simulink model "nms_sim_2D_cost"  (R2024b)
settings: Solver=ode15s  StartTime=0.0  StopTime=t_sim  MaxStep=dt_max  EnableMultiTasking=on
values from neighbouring files (symbols this model uses):
  a_BFSH = param_ctrl(35)*1    [setCtrlPar_optim_CPGreflex2001_2D.m]
  a_GAS = param_ctrl(37)*1    [setCtrlPar_optim_CPGreflex2001_2D.m]
  a_GLU = param_ctrl(31)*1    [setCtrlPar_optim_CPGreflex2001_2D.m]
  a_HAM = param_ctrl(33)*1    [setCtrlPar_optim_CPGreflex2001_2D.m]
  a_HFL = param_ctrl(32)*1    [setCtrlPar_optim_CPGreflex2001_2D.m]
  a_RF = param_ctrl(34)*1    [setCtrlPar_optim_CPGreflex2001_2D.m]
  a_SOL = param_ctrl(38)*1    [setCtrlPar_optim_CPGreflex2001_2D.m]
  a_TA = param_ctrl(39)*1    [setCtrlPar_optim_CPGreflex2001_2D.m]
  a_VAS = param_ctrl(36)*1    [setCtrlPar_optim_CPGreflex2001_2D.m]
  ai = param_ctrl(96)*2.0    [setCtrlPar_optim_CPGreflex2001_2D.m]
  b_BFSH = param_ctrl(52)*.51    [setCtrlPar_optim_CPGreflex2001_2D.m]
  b_BFSHGAS = param_ctrl(55)*.51    [setCtrlPar_optim_CPGreflex2001_2D.m]
  b_BFSHHAM = param_ctrl(54)*.51    [setCtrlPar_optim_CPGreflex2001_2D.m]
  b_BFSHVAS = param_ctrl(53)*.51    [setCtrlPar_optim_CPGreflex2001_2D.m]
  b_GAS = param_ctrl(59)*.51    [setCtrlPar_optim_CPGreflex2001_2D.m]
  b_GASBFSH = param_ctrl(60)*.51    [setCtrlPar_optim_CPGreflex2001_2D.m]
  b_GASSOL = param_ctrl(61)*.51    [setCtrlPar_optim_CPGreflex2001_2D.m]
  b_GLU = param_ctrl(40)*.51    [setCtrlPar_optim_CPGreflex2001_2D.m]
  b_GLUHAM = param_ctrl(42)*.51    [setCtrlPar_optim_CPGreflex2001_2D.m]
  b_GLUHFL = param_ctrl(41)*.51    [setCtrlPar_optim_CPGreflex2001_2D.m]
  b_HAM = param_ctrl(46)*.51    [setCtrlPar_optim_CPGreflex2001_2D.m]
  b_HAMBFSH = param_ctrl(48)*.51    [setCtrlPar_optim_CPGreflex2001_2D.m]
  b_HAMGLU = param_ctrl(47)*.51    [setCtrlPar_optim_CPGreflex2001_2D.m]
  b_HFL = param_ctrl(43)*.51    [setCtrlPar_optim_CPGreflex2001_2D.m]
  b_HFLGLU = param_ctrl(44)*.51    [setCtrlPar_optim_CPGreflex2001_2D.m]
  b_HFLRF = param_ctrl(45)*.51    [setCtrlPar_optim_CPGreflex2001_2D.m]
  b_RF = param_ctrl(49)*.51    [setCtrlPar_optim_CPGreflex2001_2D.m]
  b_RFHFL = param_ctrl(50)*.51    [setCtrlPar_optim_CPGreflex2001_2D.m]
  b_RFVAS = param_ctrl(51)*.51    [setCtrlPar_optim_CPGreflex2001_2D.m]
  b_SOL = param_ctrl(62)*.51    [setCtrlPar_optim_CPGreflex2001_2D.m]
  b_SOLGAS = param_ctrl(64)*.51    [setCtrlPar_optim_CPGreflex2001_2D.m]
  b_SOLTA = param_ctrl(63)*.51    [setCtrlPar_optim_CPGreflex2001_2D.m]
  b_TA = param_ctrl(65)*.51    [setCtrlPar_optim_CPGreflex2001_2D.m]
  b_TASOL = param_ctrl(66)*.51    [setCtrlPar_optim_CPGreflex2001_2D.m]
  b_VAS = param_ctrl(56)*.51    [setCtrlPar_optim_CPGreflex2001_2D.m]
  b_VASBFSH = param_ctrl(57)*.51    [setCtrlPar_optim_CPGreflex2001_2D.m]
  b_VASRF = param_ctrl(58)*.51    [setCtrlPar_optim_CPGreflex2001_2D.m]
  bias = param_ctrl(97)*2.5    [setCtrlPar_optim_CPGreflex2001_2D.m]
  c = 0.05    [nms_MS_2D_scaled.m]
  c_jointstop = 0.3 / (pi/180)    (= 17.1887338539)    [nms_MS_2D_scaled.m]
  D12_F = 0.16    *scaleL_JPhys    [nms_MechInit_2D_scaleSkel.m]
  D12_S = 0.2460	*sub_height    [nms_MechInit_2D_scaleSkel.m]
  D12_T = 0.2450  *sub_height    [nms_MechInit_2D_scaleSkel.m]
  D12y_F = 0.039  *sub_height    [nms_MechInit_2D_scaleSkel.m]
  D12z_HAT = 0.1    [nms_MS_2D_scaled.m]
  D13_F = 0.20    *scaleL_JPhys    [nms_MechInit_2D_scaleSkel.m]
  D1G_F = 0.14    *scaleL_JPhys    [nms_MechInit_2D_scaleSkel.m]
  D1G_HAT = 0.35  *scaleL_JPhys    [nms_MechInit_2D_scaleSkel.m]
  D1G_S = (0.3 - D12y_F/4)	*scaleL_JPhys    [nms_MechInit_2D_scaleSkel.m]
  D1G_T = (0.3 - D12y_F/4)	*scaleL_JPhys    [nms_MechInit_2D_scaleSkel.m]
  D1Gy_F = D12y_F*D1G_F/D12_F    (= 0.07)    [nms_MechInit_2D_scaleSkel.m]
  d_BFSH = param_ctrl(26)*1    [setCtrlPar_optim_CPGreflex2001_2D.m]
  d_GAS = param_ctrl(28)*1    [setCtrlPar_optim_CPGreflex2001_2D.m]
  d_GLU = param_ctrl(22)*1    [setCtrlPar_optim_CPGreflex2001_2D.m]
  d_HAM = param_ctrl(24)*1    [setCtrlPar_optim_CPGreflex2001_2D.m]
  d_HFL = param_ctrl(23)*1    [setCtrlPar_optim_CPGreflex2001_2D.m]
  d_RF = param_ctrl(25)*1    [setCtrlPar_optim_CPGreflex2001_2D.m]
  d_SOL = param_ctrl(29)*1    [setCtrlPar_optim_CPGreflex2001_2D.m]
  d_TA = param_ctrl(30)*1    [setCtrlPar_optim_CPGreflex2001_2D.m]
  d_VAS = param_ctrl(27)*1    [setCtrlPar_optim_CPGreflex2001_2D.m]
  DeltaThRef = 5e-3    (= 0.005)    [nms_MS_2D_scaled.m]
  dloptBFSH = 3.0    (= 3)    [setCtrlPar_optim_CPGreflex2001_2D.m]
  dloptGAS = 3.0    (= 3)    [setCtrlPar_optim_CPGreflex2001_2D.m]
  dloptGLU = 3.0    (= 3)    [setCtrlPar_optim_CPGreflex2001_2D.m]
  dloptHAM = 3.0    (= 3)    [setCtrlPar_optim_CPGreflex2001_2D.m]
  dloptHFL = 3.0    (= 3)    [setCtrlPar_optim_CPGreflex2001_2D.m]
  dloptRF = 3.0    (= 3)    [setCtrlPar_optim_CPGreflex2001_2D.m]
  dloptSOL = 3.0    (= 3)    [setCtrlPar_optim_CPGreflex2001_2D.m]
  dloptTA = 3.0    (= 3)    [setCtrlPar_optim_CPGreflex2001_2D.m]
  dloptVAS = 3.0    (= 3)    [setCtrlPar_optim_CPGreflex2001_2D.m]
  ec_BFSH = param_ctrl(80)*0.15    [setCtrlPar_optim_CPGreflex2001_2D.m]
  ec_GAS = param_ctrl(82)*0.15    [setCtrlPar_optim_CPGreflex2001_2D.m]
  ec_GLU = param_ctrl(76)*0.15    [setCtrlPar_optim_CPGreflex2001_2D.m]
  ec_HAM = param_ctrl(78)*0.15    [setCtrlPar_optim_CPGreflex2001_2D.m]
  ec_HFL = param_ctrl(77)*0.15    [setCtrlPar_optim_CPGreflex2001_2D.m]
  ec_RF = param_ctrl(79)*0.15    [setCtrlPar_optim_CPGreflex2001_2D.m]
  ec_TA = param_ctrl(84)*0.15    [setCtrlPar_optim_CPGreflex2001_2D.m]
  ec_VAS = param_ctrl(81)*0.15    [setCtrlPar_optim_CPGreflex2001_2D.m]
  eref = 0.04    [nms_MS_2D_scaled.m]
  eref_GAS = 0.1    [nms_MS_2D_scaled.m]
  eref_SOL = 0.1    [nms_MS_2D_scaled.m]
  es_BFSH = param_ctrl(89)*0.15    [setCtrlPar_optim_CPGreflex2001_2D.m]
  es_GAS = param_ctrl(91)*0.15    [setCtrlPar_optim_CPGreflex2001_2D.m]
  es_GLU = param_ctrl(85)*0.15    [setCtrlPar_optim_CPGreflex2001_2D.m]
  es_HAM = param_ctrl(87)*0.15    [setCtrlPar_optim_CPGreflex2001_2D.m]
  es_HFL = param_ctrl(86)*0.15    [setCtrlPar_optim_CPGreflex2001_2D.m]
  es_RF = param_ctrl(88)*0.15    [setCtrlPar_optim_CPGreflex2001_2D.m]
  es_TA = param_ctrl(93)*0.15    [setCtrlPar_optim_CPGreflex2001_2D.m]
  es_VAS = param_ctrl(90)*0.15    [setCtrlPar_optim_CPGreflex2001_2D.m]
  FmaxBFSH = 350    [nms_MS_2D_scaled.m]
  FmaxGAS = 2000    [nms_MS_2D_scaled.m]
  FmaxGLU = 4000    [nms_MS_2D_scaled.m]
  FmaxHAM = 2000    [nms_MS_2D_scaled.m]
  FmaxHFL = 2000    [nms_MS_2D_scaled.m]
  FmaxRF = 850    [nms_MS_2D_scaled.m]
  FmaxSOL = 4000    [nms_MS_2D_scaled.m]
  FmaxTA = 800    [nms_MS_2D_scaled.m]
  FmaxVAS = 5000    [nms_MS_2D_scaled.m]
  g = 9.81    [nms_MS_2D_scaled.m]
  gamma_4 = param_ctrl(11) * 1.7    [setCtrlPar_optim_CPGreflexsynergy2023_2D.m]
  h_BFSH = param_ctrl(71)*.1    [setCtrlPar_optim_CPGreflex2001_2D.m]
  h_GAS = param_ctrl(73)*.1    [setCtrlPar_optim_CPGreflex2001_2D.m]
  h_GLU = param_ctrl(67)*.1    [setCtrlPar_optim_CPGreflex2001_2D.m]
  h_HAM = param_ctrl(69)*.1    [setCtrlPar_optim_CPGreflex2001_2D.m]
  h_HFL = param_ctrl(68)*.1    [setCtrlPar_optim_CPGreflex2001_2D.m]
  h_RF = param_ctrl(70)*.1    [setCtrlPar_optim_CPGreflex2001_2D.m]
  h_SOL = param_ctrl(74)*.1    [setCtrlPar_optim_CPGreflex2001_2D.m]
  h_TA = param_ctrl(75)*.1    [setCtrlPar_optim_CPGreflex2001_2D.m]
  h_VAS = param_ctrl(72)*.1    [setCtrlPar_optim_CPGreflex2001_2D.m]
  HLCtrlPar = [theta_tgt l_clr alpha_tgt alpha_cd alpha_cv]    [setCtrlPar_optim_reflex2015_2D.m]
  In_F = 0.005    *scaleM*scaleL_JPhys^2    [nms_MechInit_2D_scaleSkel.m]
  In_HAT = 2.5    *scaleM*scaleL_JPhys^2    [nms_MechInit_2D_scaleSkel.m]
  In_S = 0.05     *scaleM*scaleL_JPhys^2    [nms_MechInit_2D_scaleSkel.m]
  In_T = 0.15     *scaleM*scaleL_JPhys^2    [nms_MechInit_2D_scaleSkel.m]
  init_exc = 0.01    [setInitPar_optim_2D.m]
  init_fm = 0.01    [setInitPar_optim_2D.m]
  init_lce = 1    [setInitPar_optim_2D.m]
  init_LCPG = param_ctrl(12) * 0.01    [setCtrlPar_optim_CPGreflexsynergy2023_2D.m]
  init_LStance = 1    [setInitPar_optim_2D.m]
  init_N1 = osc_signal1(phi_off_osc_ind)    [setCtrlPar_optim_CPGreflex2001_2D.m]
  ... (+441 more)
undefined symbols (not defined in the file or in its folder): cost_act_exponent, cost_v_tgt, flag_controller, Newton, nStep_obj, nStep_startKin, Raphson, sgn, SSW_kin, terrain_slope_angle, v_plateS1, X, Y, Z
libraries: nesl_utility x94, sm_lib x90, simulink x28, simulink_extras x12
(part 10 of 20)

== system nms_sim_2D_cost/Cost/joint overextension ==
  L ankle pain lower : Fcn  Expr=u(2) * (u(1)<0)
  L ankle pain upper : Fcn  Expr=u(2) * (u(1)>0)
  L hip pain lower : Fcn  Expr=u(2) * (u(1)<0)
  L hip pain upper : Fcn  Expr=u(2) * (u(1)>0)
  L knee pain lower : Fcn  Expr=u(2) * (u(1)<0)
  L knee pain upper : Fcn  Expr=u(2) * (u(1)>0)
  Mux{1,3,5..11,13..14,16} (12 alike) : Mux  Inputs=2
  Mux15 : Mux  Inputs=12
  R ankle pain lower : Fcn  Expr=u(2) * (u(1)<0)
  R ankle pain upper : Fcn  Expr=u(2) * (u(1)>0)
  R hip Pain Upper : Fcn  Expr=u(2) * (u(1)>0)
  R hip pain lower : Fcn  Expr=u(2) * (u(1)<0)
  R hip pain upper : Fcn  Expr=u(2) * (u(1)>0)
  R knee pain lower : Fcn  Expr=u(2) * (u(1)<0)
  Sum{1,3,5,7..15} (12 alike) : Sum  Inputs=-+|
  knee lim : Constant  Value=P_kneeUpLim
  knee lim10 : Constant  Value=P_hipUpLim
  knee lim11 : Constant  Value=P_ankleUpLim
  knee lim12 : Constant  Value=P_hipLowLim
  knee lim13 : Constant  Value=P_kneeLowLim
  knee lim14 : Constant  Value=P_ankleLowLim
  knee lim2 : Constant  Value=P_hipUpLim
  knee lim4 : Constant  Value=P_ankleUpLim
  knee lim6 : Constant  Value=P_hipLowLim
  knee lim7 : Constant  Value=P_kneeLowLim
  knee lim8 : Constant  Value=P_ankleLowLim
  knee lim9 : Constant  Value=P_kneeUpLim
  pain : Outport
  wires:
  [Rphi23] -> Sum1/2
  knee lim/1 -> Sum1/1
  R hip Pain Upper/1 -> Mux15/3
  Mux10/1 -> R hip Pain Upper/1
  [RHipStop] -> Mux1/2
  Sum1/1 -> Mux10/1
  [RKneeStop] -> Mux10/2
  Mux15/1 -> pain/1
  knee lim2/1 -> Sum3/1
  Mux1/1 -> R hip pain upper/1
  [Rphi34] -> Sum3/2
  Sum3/1 -> Mux1/1
  R hip pain upper/1 -> Mux15/1
  R ankle pain upper/1 -> Mux15/5
  Mux3/1 -> R ankle pain upper/1
  knee lim4/1 -> Sum5/1
  Sum5/1 -> Mux3/1
  [Rphi12] -> Sum5/2
  [RAnkleStop] -> Mux3/2
  R hip pain lower/1 -> Mux15/2
  Sum7/1 -> Mux5/1
  [Rphi34] -> Sum7/2
  Mux5/1 -> R hip pain lower/1
  knee lim6/1 -> Sum7/1
  [RHipStop] -> Mux5/2
  [RKneeStop] -> Mux6/2
  knee lim7/1 -> Sum8/1
  Mux6/1 -> R knee pain lower/1
  [Rphi23] -> Sum8/2
  Sum8/1 -> Mux6/1
  Sum9/1 -> Mux7/1
  [Rphi12] -> Sum9/2
  Mux7/1 -> R ankle pain lower/1
  knee lim8/1 -> Sum9/1
  [RAnkleStop] -> Mux7/2
  R knee pain lower/1 -> Mux15/4
  R ankle pain lower/1 -> Mux15/6
  [LAnkleStop] -> Mux16/2
  knee lim14/1 -> Sum15/1
  Mux16/1 -> L ankle pain lower/1
  [Lphi12] -> Sum15/2
  Sum15/1 -> Mux16/1
  Sum14/1 -> Mux14/1
  [Lphi23] -> Sum14/2
  Mux14/1 -> L knee pain lower/1
  knee lim13/1 -> Sum14/1
  [LKneeStop] -> Mux14/2
  [LHipStop] -> Mux13/2
  knee lim12/1 -> Sum13/1
  Mux13/1 -> L hip pain lower/1
  [Lphi34] -> Sum13/2
  Sum13/1 -> Mux13/1
  [LAnkleStop] -> Mux11/2
  [Lphi12] -> Sum12/2
  Sum12/1 -> Mux11/1
  knee lim11/1 -> Sum12/1
  Mux11/1 -> L ankle pain upper/1
  Sum11/1 -> Mux8/1
  [Lphi34] -> Sum11/2
  Mux8/1 -> L hip pain upper/1
  knee lim10/1 -> Sum11/1
  [LKneeStop] -> Mux9/2
  Sum10/1 -> Mux9/1
  [LHipStop] -> Mux8/2
  Mux9/1 -> L knee pain upper/1
  knee lim9/1 -> Sum10/1
  [Lphi23] -> Sum10/2
  L hip pain upper/1 -> Mux15/7
  L knee pain upper/1 -> Mux15/9
  L knee pain lower/1 -> Mux15/10
  L ankle pain upper/1 -> Mux15/11
  L ankle pain lower/1 -> Mux15/12
  L hip pain lower/1 -> Mux15/8

== system nms_sim_2D_cost/Cost/nStep start ==
  nStep : Inport
  Trigger : TriggerPort  VariantControl=Variant  ZeroCross=off
  nStep_start : Outport  InitialOutput=0
  wires:
  nStep/1 -> nStep_start/1

== system nms_sim_2D_cost/Muscle Actuation/ECC ==
  E : Inport
  Constant : Constant  Value=tau_act
  Constant1 : Constant  Value=tau_deact
  Divide : Product  Inputs=*/
  Integrator : Integrator  InitialCondition=init_exc
  Sum : Sum  Inputs=+-|
  Switch : Switch  Criteria=u2 > Threshold  SaturateOnIntegerOverflow=off  InputSameDT=off
  A : Outport  VectorParamsAs1DForOutWhenUnconnected=off
  wires:
  E/1 -> Sum/1
  Integrator/1 -> A/1, Sum/2  "A"
  Divide/1 -> Integrator/1  "dA"
  Sum/1 -> Divide/1, Switch/2
  Switch/1 -> Divide/2
  Constant/1 -> Switch/1
  Constant1/1 -> Switch/3

== system nms_sim_2D_cost/Muscle Actuation/ECC1 ==
  E : Inport
  Constant : Constant  Value=tau_act
  Constant1 : Constant  Value=tau_deact
  Divide : Product  Inputs=*/
  Integrator : Integrator  InitialCondition=init_exc
  Sum : Sum  Inputs=+-|
  Switch : Switch  Criteria=u2 > Threshold  SaturateOnIntegerOverflow=off  InputSameDT=off
  A : Outport  VectorParamsAs1DForOutWhenUnconnected=off
  wires:
  Constant1/1 -> Switch/3
  Constant/1 -> Switch/1
  Switch/1 -> Divide/2
  Sum/1 -> Switch/2, Divide/1
  Divide/1 -> Integrator/1  "dA"
  Integrator/1 -> Sum/2, A/1  "A"
  E/1 -> Sum/1

== system nms_sim_2D_cost/Muscle Actuation/ECC10 ==
  E : Inport
  Constant : Constant  Value=tau_act
  Constant1 : Constant  Value=tau_deact
  Divide : Product  Inputs=*/
  Integrator : Integrator  InitialCondition=init_exc
  Sum : Sum  Inputs=+-|
  Switch : Switch  Criteria=u2 > Threshold  SaturateOnIntegerOverflow=off  InputSameDT=off
  A : Outport  VectorParamsAs1DForOutWhenUnconnected=off
  wires:
  Constant1/1 -> Switch/3
  Constant/1 -> Switch/1
  Switch/1 -> Divide/2
  Sum/1 -> Switch/2, Divide/1
  Divide/1 -> Integrator/1  "dA"
  Integrator/1 -> Sum/2, A/1  "A"
  E/1 -> Sum/1

== system nms_sim_2D_cost/Muscle Actuation/ECC11 ==
  E : Inport
  Constant : Constant  Value=tau_act
  Constant1 : Constant  Value=tau_deact
  Divide : Product  Inputs=*/
  Integrator : Integrator  InitialCondition=init_exc
  Sum : Sum  Inputs=+-|
  Switch : Switch  Criteria=u2 > Threshold  SaturateOnIntegerOverflow=off  InputSameDT=off
  A : Outport  VectorParamsAs1DForOutWhenUnconnected=off
  wires:
  E/1 -> Sum/1
  Integrator/1 -> A/1, Sum/2  "A"
  Divide/1 -> Integrator/1  "dA"
  Sum/1 -> Divide/1, Switch/2
  Switch/1 -> Divide/2
  Constant/1 -> Switch/1
  Constant1/1 -> Switch/3

== system nms_sim_2D_cost/Muscle Actuation/ECC12 ==
  E : Inport
  Constant : Constant  Value=tau_act
  Constant1 : Constant  Value=tau_deact
  Divide : Product  Inputs=*/
  Integrator : Integrator  InitialCondition=init_exc
  Sum : Sum  Inputs=+-|
  Switch : Switch  Criteria=u2 > Threshold  SaturateOnIntegerOverflow=off  InputSameDT=off
  A : Outport  VectorParamsAs1DForOutWhenUnconnected=off
  wires:
  Constant1/1 -> Switch/3
  Constant/1 -> Switch/1
  Switch/1 -> Divide/2
  Sum/1 -> Switch/2, Divide/1
  Divide/1 -> Integrator/1  "dA"
  Integrator/1 -> Sum/2, A/1  "A"
  E/1 -> Sum/1

== system nms_sim_2D_cost/Muscle Actuation/ECC13 ==
  E : Inport
  Constant : Constant  Value=tau_act
  Constant1 : Constant  Value=tau_deact
  Divide : Product  Inputs=*/
  Integrator : Integrator  InitialCondition=init_exc
  Sum : Sum  Inputs=+-|
  Switch : Switch  Criteria=u2 > Threshold  SaturateOnIntegerOverflow=off  InputSameDT=off
  A : Outport  VectorParamsAs1DForOutWhenUnconnected=off
  wires:
  E/1 -> Sum/1
  Integrator/1 -> A/1, Sum/2  "A"
  Divide/1 -> Integrator/1  "dA"
  Sum/1 -> Divide/1, Switch/2
  Switch/1 -> Divide/2
  Constant/1 -> Switch/1
  Constant1/1 -> Switch/3

== system nms_sim_2D_cost/Muscle Actuation/ECC14 ==
  E : Inport
  Constant : Constant  Value=tau_act
  Constant1 : Constant  Value=tau_deact
  Divide : Product  Inputs=*/
  Integrator : Integrator  InitialCondition=init_exc
  Sum : Sum  Inputs=+-|
  Switch : Switch  Criteria=u2 > Threshold  SaturateOnIntegerOverflow=off  InputSameDT=off
  A : Outport  VectorParamsAs1DForOutWhenUnconnected=off
  wires:
  Constant1/1 -> Switch/3
  Constant/1 -> Switch/1
  Switch/1 -> Divide/2
  Sum/1 -> Switch/2, Divide/1
  Divide/1 -> Integrator/1  "dA"
  Integrator/1 -> Sum/2, A/1  "A"
  E/1 -> Sum/1

== system nms_sim_2D_cost/Muscle Actuation/ECC15 ==
  E : Inport
  Constant : Constant  Value=tau_act
  Constant1 : Constant  Value=tau_deact
  Divide : Product  Inputs=*/
  Integrator : Integrator  InitialCondition=init_exc
  Sum : Sum  Inputs=+-|
  Switch : Switch  Criteria=u2 > Threshold  SaturateOnIntegerOverflow=off  InputSameDT=off
  A : Outport  VectorParamsAs1DForOutWhenUnconnected=off
  wires:
  E/1 -> Sum/1
  Integrator/1 -> A/1, Sum/2  "A"
  Divide/1 -> Integrator/1  "dA"
  Sum/1 -> Divide/1, Switch/2
  Switch/1 -> Divide/2
  Constant/1 -> Switch/1
  Constant1/1 -> Switch/3

== system nms_sim_2D_cost/Muscle Actuation/ECC16 ==
  E : Inport
  Constant : Constant  Value=tau_act
  Constant1 : Constant  Value=tau_deact
  Divide : Product  Inputs=*/
  Integrator : Integrator  InitialCondition=init_exc
  Sum : Sum  Inputs=+-|
  Switch : Switch  Criteria=u2 > Threshold  SaturateOnIntegerOverflow=off  InputSameDT=off
  A : Outport  VectorParamsAs1DForOutWhenUnconnected=off
  wires:
  Constant1/1 -> Switch/3
  Constant/1 -> Switch/1
  Switch/1 -> Divide/2
  Sum/1 -> Switch/2, Divide/1
  Divide/1 -> Integrator/1  "dA"
  Integrator/1 -> Sum/2, A/1  "A"
  E/1 -> Sum/1

== system nms_sim_2D_cost/Muscle Actuation/ECC17 ==
  E : Inport
  Constant : Constant  Value=tau_act
  Constant1 : Constant  Value=tau_deact
  Divide : Product  Inputs=*/
  Integrator : Integrator  InitialCondition=init_exc
  Sum : Sum  Inputs=+-|
  Switch : Switch  Criteria=u2 > Threshold  SaturateOnIntegerOverflow=off  InputSameDT=off
  A : Outport  VectorParamsAs1DForOutWhenUnconnected=off
  wires:
  E/1 -> Sum/1
  Integrator/1 -> A/1, Sum/2  "A"
  Divide/1 -> Integrator/1  "dA"
  Sum/1 -> Divide/1, Switch/2
  Switch/1 -> Divide/2
  Constant/1 -> Switch/1
  Constant1/1 -> Switch/3

== system nms_sim_2D_cost/Muscle Actuation/ECC2 ==
  E : Inport
  Constant : Constant  Value=tau_act
  Constant1 : Constant  Value=tau_deact
  Divide : Product  Inputs=*/
  Integrator : Integrator  InitialCondition=init_exc
  Sum : Sum  Inputs=+-|
  Switch : Switch  Criteria=u2 > Threshold  SaturateOnIntegerOverflow=off  InputSameDT=off
  A : Outport  VectorParamsAs1DForOutWhenUnconnected=off
  wires:
  E/1 -> Sum/1
  Integrator/1 -> A/1, Sum/2  "A"
  Divide/1 -> Integrator/1  "dA"
  Sum/1 -> Divide/1, Switch/2
  Switch/1 -> Divide/2
  Constant/1 -> Switch/1
  Constant1/1 -> Switch/3

== system nms_sim_2D_cost/Muscle Actuation/ECC3 ==
  E : Inport
  Constant : Constant  Value=tau_act
  Constant1 : Constant  Value=tau_deact
  Divide : Product  Inputs=*/
  Integrator : Integrator  InitialCondition=init_exc
  Sum : Sum  Inputs=+-|
  Switch : Switch  Criteria=u2 > Threshold  SaturateOnIntegerOverflow=off  InputSameDT=off
  A : Outport  VectorParamsAs1DForOutWhenUnconnected=off
  wires:
  Constant1/1 -> Switch/3
  Constant/1 -> Switch/1
  Switch/1 -> Divide/2
  Sum/1 -> Switch/2, Divide/1
  Divide/1 -> Integrator/1  "dA"
  Integrator/1 -> Sum/2, A/1  "A"
  E/1 -> Sum/1

== system nms_sim_2D_cost/Muscle Actuation/ECC4 ==
  E : Inport
  Constant : Constant  Value=tau_act
  Constant1 : Constant  Value=tau_deact
  Divide : Product  Inputs=*/
  Integrator : Integrator  InitialCondition=init_exc
  Sum : Sum  Inputs=+-|
  Switch : Switch  Criteria=u2 > Threshold  SaturateOnIntegerOverflow=off  InputSameDT=off
  A : Outport  VectorParamsAs1DForOutWhenUnconnected=off
  wires:
  E/1 -> Sum/1
  Integrator/1 -> A/1, Sum/2  "A"
  Divide/1 -> Integrator/1  "dA"
  Sum/1 -> Divide/1, Switch/2
  Switch/1 -> Divide/2
  Constant/1 -> Switch/1
  Constant1/1 -> Switch/3

== system nms_sim_2D_cost/Muscle Actuation/ECC5 ==
  E : Inport
  Constant : Constant  Value=tau_act
  Constant1 : Constant  Value=tau_deact
  Divide : Product  Inputs=*/
  Integrator : Integrator  InitialCondition=init_exc
  Sum : Sum  Inputs=+-|
  Switch : Switch  Criteria=u2 > Threshold  SaturateOnIntegerOverflow=off  InputSameDT=off
  A : Outport  VectorParamsAs1DForOutWhenUnconnected=off
  wires:
  Constant1/1 -> Switch/3
  Constant/1 -> Switch/1
  Switch/1 -> Divide/2
  Sum/1 -> Switch/2, Divide/1
  Divide/1 -> Integrator/1  "dA"
  Integrator/1 -> Sum/2, A/1  "A"
  E/1 -> Sum/1

== system nms_sim_2D_cost/Muscle Actuation/ECC6 ==
  E : Inport
  Constant : Constant  Value=tau_act
  Constant1 : Constant  Value=tau_deact
  Divide : Product  Inputs=*/
  Integrator : Integrator  InitialCondition=init_exc
  Sum : Sum  Inputs=+-|
  Switch : Switch  Criteria=u2 > Threshold  SaturateOnIntegerOverflow=off  InputSameDT=off
  A : Outport  VectorParamsAs1DForOutWhenUnconnected=off
  wires:
  E/1 -> Sum/1
  Integrator/1 -> A/1, Sum/2  "A"
  Divide/1 -> Integrator/1  "dA"
  Sum/1 -> Divide/1, Switch/2
  Switch/1 -> Divide/2
  Constant/1 -> Switch/1
  Constant1/1 -> Switch/3

== system nms_sim_2D_cost/Muscle Actuation/ECC7 ==
  E : Inport
  Constant : Constant  Value=tau_act
  Constant1 : Constant  Value=tau_deact
  Divide : Product  Inputs=*/
  Integrator : Integrator  InitialCondition=init_exc
  Sum : Sum  Inputs=+-|
  Switch : Switch  Criteria=u2 > Threshold  SaturateOnIntegerOverflow=off  InputSameDT=off
  A : Outport  VectorParamsAs1DForOutWhenUnconnected=off
  wires:
  Constant1/1 -> Switch/3
  Constant/1 -> Switch/1
  Switch/1 -> Divide/2
  Sum/1 -> Switch/2, Divide/1
  Divide/1 -> Integrator/1  "dA"
  Integrator/1 -> Sum/2, A/1  "A"
  E/1 -> Sum/1

== system nms_sim_2D_cost/Muscle Actuation/ECC8 ==
  E : Inport
  Constant : Constant  Value=tau_act
  Constant1 : Constant  Value=tau_deact
  Divide : Product  Inputs=*/
  Integrator : Integrator  InitialCondition=init_exc
  Sum : Sum  Inputs=+-|
  Switch : Switch  Criteria=u2 > Threshold  SaturateOnIntegerOverflow=off  InputSameDT=off
  A : Outport  VectorParamsAs1DForOutWhenUnconnected=off
  wires:
  E/1 -> Sum/1
  Integrator/1 -> A/1, Sum/2  "A"
  Divide/1 -> Integrator/1  "dA"
  Sum/1 -> Divide/1, Switch/2
  Switch/1 -> Divide/2
  Constant/1 -> Switch/1
  Constant1/1 -> Switch/3

== system nms_sim_2D_cost/Muscle Actuation/ECC9 ==
  E : Inport
  Constant : Constant  Value=tau_act
  Constant1 : Constant  Value=tau_deact
  Divide : Product  Inputs=*/
  Integrator : Integrator  InitialCondition=init_exc
  Sum : Sum  Inputs=+-|
  Switch : Switch  Criteria=u2 > Threshold  SaturateOnIntegerOverflow=off  InputSameDT=off
  A : Outport  VectorParamsAs1DForOutWhenUnconnected=off
  wires:
  E/1 -> Sum/1
  Integrator/1 -> A/1, Sum/2  "A"
  Divide/1 -> Integrator/1  "dA"
  Sum/1 -> Divide/1, Switch/2
  Switch/1 -> Divide/2
  Constant/1 -> Switch/1
  Constant1/1 -> Switch/3

== system nms_sim_2D_cost/Muscle Actuation/GLU ==
  note: SOLEUS Muscle-Tendon Dynamics
  note: Excitation Contraction Coupling
  A : Inport
  lmtc [m] : Inport  Port=2
  1 : Product  Inputs=**  InputSameDT=on  SaturateOnIntegerOverflow=on  OutDataTypeStr=Inherit: Same as first input
  1/lslack : Gain  Gain=1/lslackGLU  SaturateOnIntegerOverflow=on  OutDataTypeStr=Inherit: Same as input  ParamDataTypeStr=Inherit: Same as input
  BE force-length relation : Subsystem
  CE force-length relation : Subsystem
  CE inverse force-velocity relation : Subsystem
  Constant : Constant  Value=lslackGLU
  Fmax : Gain  Gain=FmaxGLU  SaturateOnIntegerOverflow=on  OutDataTypeStr=Inherit: Same as input  ParamDataTypeStr=Inherit: Same as input
  Fmax1 : Gain  Gain=FmaxGLU  SaturateOnIntegerOverflow=on  OutDataTypeStr=Inherit: Same as input  ParamDataTypeStr=Inherit: Same as input
  "Fpe = F^*pe * fv " : Product  InputSameDT=on  SaturateOnIntegerOverflow=on  OutDataTypeStr=Inherit: Same as first input
  Fv = Fse / (A*Fce) : Product  Inputs=*/  InputSameDT=on  SaturateOnIntegerOverflow=on  OutDataTypeStr=Inherit: Same as first input
  Integrator : Integrator  InitialConditionSource=external  LowerSaturationLimit=0.05
  PE force-length relation : Subsystem
  SE force-length relation : Subsystem
  Sum : Sum  Inputs=|+-  InputSameDT=on  SaturateOnIntegerOverflow=on  OutDataTypeStr=Inherit: Same as first input
  Sum1 : Sum  Inputs=|+-  InputSameDT=on  SaturateOnIntegerOverflow=on  OutDataTypeStr=Inherit: Same as first input
  Sum2 : Sum  Inputs=|-+  InputSameDT=on  SaturateOnIntegerOverflow=on  OutDataTypeStr=Inherit: Same as first input
  Sum3 : Sum  InputSameDT=on  SaturateOnIntegerOverflow=on  OutDataTypeStr=Inherit: Same as first input
  Sum4 : Sum  InputSameDT=on  SaturateOnIntegerOverflow=on  OutDataTypeStr=Inherit: Same as first input
  lce/lopt : Gain  Gain=1/loptGLU  SaturateOnIntegerOverflow=on  OutDataTypeStr=Inherit: Same as input  ParamDataTypeStr=Inherit: Same as input
  vmax*lopt : Gain  Gain=vmaxGLU*loptGLU  SaturateOnIntegerOverflow=on  OutDataTypeStr=Inherit: Same as input  ParamDataTypeStr=Inherit: Same as input
  Fmtc : Outport  InitialOutput=0  VectorParamsAs1DForOutWhenUnconnected=off
  Lce : Outport  Port=2  InitialOutput=0  VectorParamsAs1DForOutWhenUnconnected=off
  Vce : Outport  Port=3  InitialOutput=0  VectorParamsAs1DForOutWhenUnconnected=off
  Fce : Outport  Port=4  InitialOutput=0  VectorParamsAs1DForOutWhenUnconnected=off
  lse [m] : Outport  Port=5  InitialOutput=0  VectorParamsAs1DForOutWhenUnconnected=off
  wires:
  Integrator/1 -> Sum/2, lce/lopt/1, Lce/1  "lce"
  Sum/1 -> lse [m]/1, 1/lslack/1  "lse"
  lce/lopt/1 -> CE force-length relation/1(lce [lopt]), BE force-length relation/1(lce [lopt]), PE force-length relation/1(lce [lopt])
  Fv = Fse / (A*Fce)/1 -> CE inverse force-velocity relation/1(Fv[Fmax]), "Fpe = F^*pe * fv "/1  "fv"
  vmax*lopt/1 -> Integrator/1, Vce/1  "vce"
  lmtc [m]/1 -> Sum2/2, Sum/1  "lmtc"
  Fmax/1 -> Fmtc/1  "Fmtc"
  1/lslack/1 -> SE force-length relation/1(lse [lslack])
  SE force-length relation/1(fse [Fmax]) -> Fmax/1, Sum4/1
  Sum2/1 -> Integrator/2
  Constant/1 -> Sum2/1
  CE force-length relation/1(fce [Fmax]) -> 1/1
  Sum4/1 -> Fv = Fse / (A*Fce)/1, Sum1/1  "Fse+Fbe"
  PE force-length relation/1(fpe [Fmax]) -> Sum3/1, "Fpe = F^*pe * fv "/2
  1/1 -> Sum3/2
  BE force-length relation/1(fbe [Fmax]) -> Sum4/2
  Sum3/1 -> Fv = Fse / (A*Fce)/2
  CE inverse force-velocity relation/1(v[vmax]) -> vmax*lopt/1
  A/1 -> 1/2
  "Fpe = F^*pe * fv "/1 -> Sum1/2
  Sum1/1 -> Fmax1/1  "Fse+Fbe-Fpe"
  Fmax1/1 -> Fce/1

== system nms_sim_2D_cost/Muscle Actuation/GLU Link ==
  note: GLUTEUS Attachment
  phi34 [rad] : Inport
  Constant : Constant  Value=lslackGLU+loptGLU
  Constant1 : Constant  Value=rGLU
  Constant2 : Constant  Value=phirefGLU
  Gain2 : Gain  Gain=rhoGLU
  Product : Product  RndMeth=Zero
  Sum2 : Sum  Inputs=|+-
  Sum5 : Sum  Inputs=|+-
  lmtu [m] : Outport  VectorParamsAs1DForOutWhenUnconnected=off
  lever [m] : Outport  Port=2  VectorParamsAs1DForOutWhenUnconnected=off
  wires:
  Constant/1 -> Sum5/1
  Sum5/1 -> lmtu [m]/1
  Product/1 -> Gain2/1
  phi34 [rad]/1 -> Sum2/1
  Constant2/1 -> Sum2/2
  Sum2/1 -> Product/1
  Constant1/1 -> Product/2, lever [m]/1
  Gain2/1 -> Sum5/2

== system nms_sim_2D_cost/Muscle Actuation/GLU1 ==
  note: SOLEUS Muscle-Tendon Dynamics
  note: Excitation Contraction Coupling
  A : Inport
  lmtc [m] : Inport  Port=2
  1 : Product  Inputs=**  InputSameDT=on  SaturateOnIntegerOverflow=on  OutDataTypeStr=Inherit: Same as first input
  1/lslack : Gain  Gain=1/lslackGLU  SaturateOnIntegerOverflow=on  OutDataTypeStr=Inherit: Same as input  ParamDataTypeStr=Inherit: Same as input
  BE force-length relation : Subsystem
  CE force-length relation : Subsystem
  CE inverse force-velocity relation : Subsystem
  Constant : Constant  Value=lslackGLU
  Fmax : Gain  Gain=FmaxGLU  SaturateOnIntegerOverflow=on  OutDataTypeStr=Inherit: Same as input  ParamDataTypeStr=Inherit: Same as input
  Fmax1 : Gain  Gain=FmaxGLU  SaturateOnIntegerOverflow=on  OutDataTypeStr=Inherit: Same as input  ParamDataTypeStr=Inherit: Same as input
  "Fpe = F^*pe * fv " : Product  InputSameDT=on  SaturateOnIntegerOverflow=on  OutDataTypeStr=Inherit: Same as first input
  Fv = Fse / (A*Fce) : Product  Inputs=*/  InputSameDT=on  SaturateOnIntegerOverflow=on  OutDataTypeStr=Inherit: Same as first input
  Integrator : Integrator  InitialConditionSource=external  LowerSaturationLimit=0.05
  PE force-length relation : Subsystem
  SE force-length relation : Subsystem
  Sum : Sum  Inputs=|+-  InputSameDT=on  SaturateOnIntegerOverflow=on  OutDataTypeStr=Inherit: Same as first input
  Sum1 : Sum  Inputs=|+-  InputSameDT=on  SaturateOnIntegerOverflow=on  OutDataTypeStr=Inherit: Same as first input
  Sum2 : Sum  Inputs=|-+  InputSameDT=on  SaturateOnIntegerOverflow=on  OutDataTypeStr=Inherit: Same as first input
  Sum3 : Sum  InputSameDT=on  SaturateOnIntegerOverflow=on  OutDataTypeStr=Inherit: Same as first input
  Sum4 : Sum  InputSameDT=on  SaturateOnIntegerOverflow=on  OutDataTypeStr=Inherit: Same as first input
  lce/lopt : Gain  Gain=1/loptGLU  SaturateOnIntegerOverflow=on  OutDataTypeStr=Inherit: Same as input  ParamDataTypeStr=Inherit: Same as input
  vmax*lopt : Gain  Gain=vmaxGLU*loptGLU  SaturateOnIntegerOverflow=on  OutDataTypeStr=Inherit: Same as input  ParamDataTypeStr=Inherit: Same as input
  Fmtc : Outport  InitialOutput=0  VectorParamsAs1DForOutWhenUnconnected=off
  Lce : Outport  Port=2  InitialOutput=0  VectorParamsAs1DForOutWhenUnconnected=off
  Vce : Outport  Port=3  InitialOutput=0  VectorParamsAs1DForOutWhenUnconnected=off
  Fce : Outport  Port=4  InitialOutput=0  VectorParamsAs1DForOutWhenUnconnected=off
  lse [m] : Outport  Port=5  InitialOutput=0  VectorParamsAs1DForOutWhenUnconnected=off
  wires:
  Integrator/1 -> Sum/2, lce/lopt/1, Lce/1  "lce"
  lce/lopt/1 -> CE force-length relation/1(lce [lopt]), PE force-length relation/1(lce [lopt]), BE force-length relation/1(lce [lopt])
  Fv = Fse / (A*Fce)/1 -> "Fpe = F^*pe * fv "/1, CE inverse force-velocity relation/1(Fv[Fmax])  "fv"
  vmax*lopt/1 -> Integrator/1, Vce/1  "vce"
  lmtc [m]/1 -> Sum2/2, Sum/1  "lmtc"
  Fmax/1 -> Fmtc/1  "Fmtc"
  1/lslack/1 -> SE force-length relation/1(lse [lslack])
  SE force-length relation/1(fse [Fmax]) -> Fmax/1, Sum4/1
  Sum2/1 -> Integrator/2
  Constant/1 -> Sum2/1
  CE force-length relation/1(fce [Fmax]) -> 1/1
  PE force-length relation/1(fpe [Fmax]) -> "Fpe = F^*pe * fv "/2, Sum3/1
  1/1 -> Sum3/2
  BE force-length relation/1(fbe [Fmax]) -> Sum4/2
  Sum3/1 -> Fv = Fse / (A*Fce)/2
  CE inverse force-velocity relation/1(v[vmax]) -> vmax*lopt/1
  A/1 -> 1/2
  Sum4/1 -> Sum1/1, Fv = Fse / (A*Fce)/1  "Fse+Fbe"
  "Fpe = F^*pe * fv "/1 -> Sum1/2
  Sum1/1 -> Fmax1/1  "Fse+Fbe-Fpe"
  Fmax1/1 -> Fce/1
  Sum/1 -> lse [m]/1, 1/lslack/1  "lse"

== system nms_sim_2D_cost/Muscle Actuation/HAM ==
  note: SOLEUS Muscle-Tendon Dynamics
  note: Excitation Contraction Coupling
  A : Inport
  lmtc [m] : Inport  Port=2
  1 : Product  Inputs=**  InputSameDT=on  SaturateOnIntegerOverflow=on  OutDataTypeStr=Inherit: Same as first input
  1/lslack : Gain  Gain=1/lslackHAM  SaturateOnIntegerOverflow=on  OutDataTypeStr=Inherit: Same as input  ParamDataTypeStr=Inherit: Same as input
  BE force-length relation : Subsystem
  CE force-length relation : Subsystem
  CE inverse force-velocity relation : Subsystem
  Constant : Constant  Value=lslackHAM
  Fmax : Gain  Gain=FmaxHAM  SaturateOnIntegerOverflow=on  OutDataTypeStr=Inherit: Same as input  ParamDataTypeStr=Inherit: Same as input
  Fmax1 : Gain  Gain=FmaxHAM  SaturateOnIntegerOverflow=on  OutDataTypeStr=Inherit: Same as input  ParamDataTypeStr=Inherit: Same as input
  "Fpe = F^*pe * fv " : Product  InputSameDT=on  SaturateOnIntegerOverflow=on  OutDataTypeStr=Inherit: Same as first input
  Fv = Fse / (A*Fce) : Product  Inputs=*/  InputSameDT=on  SaturateOnIntegerOverflow=on  OutDataTypeStr=Inherit: Same as first input
  Integrator : Integrator  InitialConditionSource=external  LowerSaturationLimit=0.05
  PE force-length relation : Subsystem
  SE force-length relation : Subsystem
  Sum : Sum  Inputs=|+-  InputSameDT=on  SaturateOnIntegerOverflow=on  OutDataTypeStr=Inherit: Same as first input
  Sum1 : Sum  Inputs=|+-  InputSameDT=on  SaturateOnIntegerOverflow=on  OutDataTypeStr=Inherit: Same as first input
  Sum2 : Sum  Inputs=|-+  InputSameDT=on  SaturateOnIntegerOverflow=on  OutDataTypeStr=Inherit: Same as first input
  Sum3 : Sum  InputSameDT=on  SaturateOnIntegerOverflow=on  OutDataTypeStr=Inherit: Same as first input
  Sum4 : Sum  InputSameDT=on  SaturateOnIntegerOverflow=on  OutDataTypeStr=Inherit: Same as first input
  lce/lopt : Gain  Gain=1/loptHAM  SaturateOnIntegerOverflow=on  OutDataTypeStr=Inherit: Same as input  ParamDataTypeStr=Inherit: Same as input
  vmax*lopt : Gain  Gain=vmaxHAM*loptHAM  SaturateOnIntegerOverflow=on  OutDataTypeStr=Inherit: Same as input  ParamDataTypeStr=Inherit: Same as input
  Fmtc : Outport  InitialOutput=0  VectorParamsAs1DForOutWhenUnconnected=off
  Lce : Outport  Port=2  InitialOutput=0  VectorParamsAs1DForOutWhenUnconnected=off
  Vce : Outport  Port=3  InitialOutput=0  VectorParamsAs1DForOutWhenUnconnected=off
  Fce : Outport  Port=4  InitialOutput=0  VectorParamsAs1DForOutWhenUnconnected=off
  lse [m] : Outport  Port=5  InitialOutput=0  VectorParamsAs1DForOutWhenUnconnected=off
  wires:
  Integrator/1 -> Sum/2, lce/lopt/1, Lce/1  "lce"
  lce/lopt/1 -> CE force-length relation/1(lce [lopt]), PE force-length relation/1(lce [lopt]), BE force-length relation/1(lce [lopt])
  Fv = Fse / (A*Fce)/1 -> "Fpe = F^*pe * fv "/1, CE inverse force-velocity relation/1(Fv[Fmax])  "fv"
  vmax*lopt/1 -> Integrator/1, Vce/1  "vce"
  lmtc [m]/1 -> Sum2/2, Sum/1  "lmtc"
  Fmax/1 -> Fmtc/1  "Fmtc"
  1/lslack/1 -> SE force-length relation/1(lse [lslack])
  SE force-length relation/1(fse [Fmax]) -> Fmax/1, Sum4/1
  Sum2/1 -> Integrator/2
  Constant/1 -> Sum2/1
  CE force-length relation/1(fce [Fmax]) -> 1/1
  PE force-length relation/1(fpe [Fmax]) -> "Fpe = F^*pe * fv "/2, Sum3/1
  1/1 -> Sum3/2
  BE force-length relation/1(fbe [Fmax]) -> Sum4/2
  Sum3/1 -> Fv = Fse / (A*Fce)/2
  CE inverse force-velocity relation/1(v[vmax]) -> vmax*lopt/1
  A/1 -> 1/2
  Sum4/1 -> Sum1/1, Fv = Fse / (A*Fce)/1  "Fse+Fbe"
  "Fpe = F^*pe * fv "/1 -> Sum1/2
  Sum1/1 -> Fmax1/1  "Fse+Fbe-Fpe"
  Fmax1/1 -> Fce/1
  Sum/1 -> lse [m]/1, 1/lslack/1  "lse"

== system nms_sim_2D_cost/Muscle Actuation/HAM Link ==
  note: HAM Attachment
  phi34 [rad] : Inport
  phi23 [rad] : Inport  Port=2
  Constant1 : Constant  Value=rHAMk
  Constant2 : Constant  Value=phirefHAMk
  Constant3 : Constant  Value=rHAMh
  Constant4 : Constant  Value=lslackHAM+loptHAM
  Constant5 : Constant  Value=phirefHAMh
  Gain2 : Gain  Gain=rhoHAMh
  Gain4 : Gain  Gain=rhoHAMk
  Product : Product  RndMeth=Zero
  Product1 : Product  RndMeth=Zero
  Sum1 : Sum  Inputs=|+-
  Sum4 : Sum  Inputs=|+-
  Sum5 : Sum  Inputs=-++
  lmtu [m] : Outport  VectorParamsAs1DForOutWhenUnconnected=off
  lever34 [m] : Outport  Port=2  VectorParamsAs1DForOutWhenUnconnected=off
  lever23 [m] : Outport  Port=3  VectorParamsAs1DForOutWhenUnconnected=off
  wires:
  Sum5/1 -> lmtu [m]/1
  Constant4/1 -> Sum5/2
  Gain4/1 -> Sum5/3
  Gain2/1 -> Sum5/1
  phi34 [rad]/1 -> Sum4/1
  Constant5/1 -> Sum4/2
  Sum4/1 -> Product/1
  Constant3/1 -> Product/2, lever34 [m]/1
  Product/1 -> Gain2/1
  phi23 [rad]/1 -> Sum1/1
  Constant2/1 -> Sum1/2
  Sum1/1 -> Product1/1
  Constant1/1 -> Product1/2, lever23 [m]/1
  Product1/1 -> Gain4/1

== system nms_sim_2D_cost/Muscle Actuation/HAM1 ==
  note: SOLEUS Muscle-Tendon Dynamics
  note: Excitation Contraction Coupling
  A : Inport
  lmtc [m] : Inport  Port=2
  1 : Product  Inputs=**  InputSameDT=on  SaturateOnIntegerOverflow=on  OutDataTypeStr=Inherit: Same as first input
  1/lslack : Gain  Gain=1/lslackHAM  SaturateOnIntegerOverflow=on  OutDataTypeStr=Inherit: Same as input  ParamDataTypeStr=Inherit: Same as input
  BE force-length relation : Subsystem
  CE force-length relation : Subsystem
  CE inverse force-velocity relation : Subsystem
  Constant : Constant  Value=lslackHAM
  Fmax : Gain  Gain=FmaxHAM  SaturateOnIntegerOverflow=on  OutDataTypeStr=Inherit: Same as input  ParamDataTypeStr=Inherit: Same as input
  Fmax1 : Gain  Gain=FmaxHAM  SaturateOnIntegerOverflow=on  OutDataTypeStr=Inherit: Same as input  ParamDataTypeStr=Inherit: Same as input
  "Fpe = F^*pe * fv " : Product  InputSameDT=on  SaturateOnIntegerOverflow=on  OutDataTypeStr=Inherit: Same as first input
  Fv = Fse / (A*Fce) : Product  Inputs=*/  InputSameDT=on  SaturateOnIntegerOverflow=on  OutDataTypeStr=Inherit: Same as first input
  Integrator : Integrator  InitialConditionSource=external  LowerSaturationLimit=0.05
  PE force-length relation : Subsystem
  SE force-length relation : Subsystem
  Sum : Sum  Inputs=|+-  InputSameDT=on  SaturateOnIntegerOverflow=on  OutDataTypeStr=Inherit: Same as first input
  Sum1 : Sum  Inputs=|+-  InputSameDT=on  SaturateOnIntegerOverflow=on  OutDataTypeStr=Inherit: Same as first input
  Sum2 : Sum  Inputs=|-+  InputSameDT=on  SaturateOnIntegerOverflow=on  OutDataTypeStr=Inherit: Same as first input
  Sum3 : Sum  InputSameDT=on  SaturateOnIntegerOverflow=on  OutDataTypeStr=Inherit: Same as first input
  Sum4 : Sum  InputSameDT=on  SaturateOnIntegerOverflow=on  OutDataTypeStr=Inherit: Same as first input
  lce/lopt : Gain  Gain=1/loptHAM  SaturateOnIntegerOverflow=on  OutDataTypeStr=Inherit: Same as input  ParamDataTypeStr=Inherit: Same as input
  vmax*lopt : Gain  Gain=vmaxHAM*loptHAM  SaturateOnIntegerOverflow=on  OutDataTypeStr=Inherit: Same as input  ParamDataTypeStr=Inherit: Same as input
  Fmtc : Outport  InitialOutput=0  VectorParamsAs1DForOutWhenUnconnected=off
  Lce : Outport  Port=2  InitialOutput=0  VectorParamsAs1DForOutWhenUnconnected=off
  Vce : Outport  Port=3  InitialOutput=0  VectorParamsAs1DForOutWhenUnconnected=off
  Fce : Outport  Port=4  InitialOutput=0  VectorParamsAs1DForOutWhenUnconnected=off
  lse [m] : Outport  Port=5  InitialOutput=0  VectorParamsAs1DForOutWhenUnconnected=off
  wires:
  Integrator/1 -> Sum/2, lce/lopt/1, Lce/1  "lce"
  lce/lopt/1 -> CE force-length relation/1(lce [lopt]), PE force-length relation/1(lce [lopt]), BE force-length relation/1(lce [lopt])
  Fv = Fse / (A*Fce)/1 -> "Fpe = F^*pe * fv "/1, CE inverse force-velocity relation/1(Fv[Fmax])  "fv"
  vmax*lopt/1 -> Integrator/1, Vce/1  "vce"
  lmtc [m]/1 -> Sum2/2, Sum/1  "lmtc"
  Fmax/1 -> Fmtc/1  "Fmtc"
  1/lslack/1 -> SE force-length relation/1(lse [lslack])
  SE force-length relation/1(fse [Fmax]) -> Fmax/1, Sum4/1
  Sum2/1 -> Integrator/2
  Constant/1 -> Sum2/1
  CE force-length relation/1(fce [Fmax]) -> 1/1
  PE force-length relation/1(fpe [Fmax]) -> "Fpe = F^*pe * fv "/2, Sum3/1
  1/1 -> Sum3/2
  BE force-length relation/1(fbe [Fmax]) -> Sum4/2
  Sum3/1 -> Fv = Fse / (A*Fce)/2
  CE inverse force-velocity relation/1(v[vmax]) -> vmax*lopt/1
  A/1 -> 1/2
  Sum4/1 -> Sum1/1, Fv = Fse / (A*Fce)/1  "Fse+Fbe"
  "Fpe = F^*pe * fv "/1 -> Sum1/2
  Sum1/1 -> Fmax1/1  "Fse+Fbe-Fpe"
  Fmax1/1 -> Fce/1
  Sum/1 -> lse [m]/1, 1/lslack/1  "lse"

== system nms_sim_2D_cost/Muscle Actuation/HFL ==
  note: SOLEUS Muscle-Tendon Dynamics
  note: Excitation Contraction Coupling
  A : Inport
  lmtc [m] : Inport  Port=2
  1 : Product  Inputs=**  InputSameDT=on  SaturateOnIntegerOverflow=on  OutDataTypeStr=Inherit: Same as first input
  1/lslack : Gain  Gain=1/lslackHFL  SaturateOnIntegerOverflow=on  OutDataTypeStr=Inherit: Same as input  ParamDataTypeStr=Inherit: Same as input
  BE force-length relation : Subsystem
  CE force-length relation : Subsystem
  CE inverse force-velocity relation : Subsystem
  Constant : Constant  Value=lslackHFL
  Fmax : Gain  Gain=FmaxHFL  SaturateOnIntegerOverflow=on  OutDataTypeStr=Inherit: Same as input  ParamDataTypeStr=Inherit: Same as input
  Fmax1 : Gain  Gain=FmaxHFL  SaturateOnIntegerOverflow=on  OutDataTypeStr=Inherit: Same as input  ParamDataTypeStr=Inherit: Same as input
  "Fpe = F^*pe * fv " : Product  InputSameDT=on  SaturateOnIntegerOverflow=on  OutDataTypeStr=Inherit: Same as first input
  Fv = Fse / (A*Fce) : Product  Inputs=*/  InputSameDT=on  SaturateOnIntegerOverflow=on  OutDataTypeStr=Inherit: Same as first input
  Integrator : Integrator  InitialConditionSource=external  LowerSaturationLimit=0.05
  PE force-length relation : Subsystem
  SE force-length relation : Subsystem
  Sum : Sum  Inputs=|+-  InputSameDT=on  SaturateOnIntegerOverflow=on  OutDataTypeStr=Inherit: Same as first input
  Sum1 : Sum  Inputs=|+-  InputSameDT=on  SaturateOnIntegerOverflow=on  OutDataTypeStr=Inherit: Same as first input
  Sum2 : Sum  Inputs=|-+  InputSameDT=on  SaturateOnIntegerOverflow=on  OutDataTypeStr=Inherit: Same as first input
  Sum3 : Sum  InputSameDT=on  SaturateOnIntegerOverflow=on  OutDataTypeStr=Inherit: Same as first input
  Sum4 : Sum  InputSameDT=on  SaturateOnIntegerOverflow=on  OutDataTypeStr=Inherit: Same as first input
  lce/lopt : Gain  Gain=1/loptHFL  SaturateOnIntegerOverflow=on  OutDataTypeStr=Inherit: Same as input  ParamDataTypeStr=Inherit: Same as input
  vmax*lopt : Gain  Gain=vmaxHFL*loptHFL  SaturateOnIntegerOverflow=on  OutDataTypeStr=Inherit: Same as input  ParamDataTypeStr=Inherit: Same as input
  Fmtc : Outport  InitialOutput=0  VectorParamsAs1DForOutWhenUnconnected=off
  Lce : Outport  Port=2  InitialOutput=0  VectorParamsAs1DForOutWhenUnconnected=off
  Vce : Outport  Port=3  InitialOutput=0  VectorParamsAs1DForOutWhenUnconnected=off
  Fce : Outport  Port=4  InitialOutput=0  VectorParamsAs1DForOutWhenUnconnected=off
  lse [m] : Outport  Port=5  InitialOutput=0  VectorParamsAs1DForOutWhenUnconnected=off
  wires:
  Integrator/1 -> Sum/2, lce/lopt/1, Lce/1  "lce"
  lce/lopt/1 -> CE force-length relation/1(lce [lopt]), PE force-length relation/1(lce [lopt]), BE force-length relation/1(lce [lopt])
  Fv = Fse / (A*Fce)/1 -> "Fpe = F^*pe * fv "/1, CE inverse force-velocity relation/1(Fv[Fmax])  "fv"
  vmax*lopt/1 -> Integrator/1, Vce/1  "vce"
  lmtc [m]/1 -> Sum2/2, Sum/1  "lmtc"
  Fmax/1 -> Fmtc/1  "Fmtc"
  1/lslack/1 -> SE force-length relation/1(lse [lslack])
  SE force-length relation/1(fse [Fmax]) -> Fmax/1, Sum4/1
  Sum2/1 -> Integrator/2
  Constant/1 -> Sum2/1
  CE force-length relation/1(fce [Fmax]) -> 1/1
  PE force-length relation/1(fpe [Fmax]) -> "Fpe = F^*pe * fv "/2, Sum3/1
  1/1 -> Sum3/2
  BE force-length relation/1(fbe [Fmax]) -> Sum4/2
  Sum3/1 -> Fv = Fse / (A*Fce)/2
  CE inverse force-velocity relation/1(v[vmax]) -> vmax*lopt/1
  A/1 -> 1/2
  Sum4/1 -> Sum1/1, Fv = Fse / (A*Fce)/1  "Fse+Fbe"
  "Fpe = F^*pe * fv "/1 -> Sum1/2
  Sum1/1 -> Fmax1/1  "Fse+Fbe-Fpe"
  Fmax1/1 -> Fce/1
  Sum/1 -> lse [m]/1, 1/lslack/1  "lse"

== system nms_sim_2D_cost/Muscle Actuation/HFL Link ==
  note: HFL Attachment
  phi34 [rad] : Inport
  Constant : Constant  Value=lslackHFL+loptHFL
  Constant1 : Constant  Value=rHFL
  Constant2 : Constant  Value=phirefHFL
  Gain2 : Gain  Gain=rhoHFL
  Product : Product  RndMeth=Zero
  Sum2 : Sum  Inputs=|+-
  Sum5 : Sum  Inputs=|++
  lmtu [m] : Outport  VectorParamsAs1DForOutWhenUnconnected=off
  lever [m] : Outport  Port=2  VectorParamsAs1DForOutWhenUnconnected=off
  wires:
  Constant/1 -> Sum5/1
  Sum5/1 -> lmtu [m]/1
  Product/1 -> Gain2/1
  phi34 [rad]/1 -> Sum2/1
  Constant2/1 -> Sum2/2
  Sum2/1 -> Product/1
  Constant1/1 -> Product/2, lever [m]/1
  Gain2/1 -> Sum5/2

== system nms_sim_2D_cost/Muscle Actuation/HFL1 ==
  note: SOLEUS Muscle-Tendon Dynamics
  note: Excitation Contraction Coupling
  A : Inport
  lmtc [m] : Inport  Port=2
  1 : Product  Inputs=**  InputSameDT=on  SaturateOnIntegerOverflow=on  OutDataTypeStr=Inherit: Same as first input
  1/lslack : Gain  Gain=1/lslackHFL  SaturateOnIntegerOverflow=on  OutDataTypeStr=Inherit: Same as input  ParamDataTypeStr=Inherit: Same as input
  BE force-length relation : Subsystem
  CE force-length relation : Subsystem
  CE inverse force-velocity relation : Subsystem
  Constant : Constant  Value=lslackHFL
  Fmax : Gain  Gain=FmaxHFL  SaturateOnIntegerOverflow=on  OutDataTypeStr=Inherit: Same as input  ParamDataTypeStr=Inherit: Same as input
  Fmax1 : Gain  Gain=FmaxHFL  SaturateOnIntegerOverflow=on  OutDataTypeStr=Inherit: Same as input  ParamDataTypeStr=Inherit: Same as input
  "Fpe = F^*pe * fv " : Product  InputSameDT=on  SaturateOnIntegerOverflow=on  OutDataTypeStr=Inherit: Same as first input
  Fv = Fse / (A*Fce) : Product  Inputs=*/  InputSameDT=on  SaturateOnIntegerOverflow=on  OutDataTypeStr=Inherit: Same as first input
  Integrator : Integrator  InitialConditionSource=external  LowerSaturationLimit=0.05
  PE force-length relation : Subsystem
  SE force-length relation : Subsystem
  Sum : Sum  Inputs=|+-  InputSameDT=on  SaturateOnIntegerOverflow=on  OutDataTypeStr=Inherit: Same as first input
  Sum1 : Sum  Inputs=|+-  InputSameDT=on  SaturateOnIntegerOverflow=on  OutDataTypeStr=Inherit: Same as first input
  Sum2 : Sum  Inputs=|-+  InputSameDT=on  SaturateOnIntegerOverflow=on  OutDataTypeStr=Inherit: Same as first input
  Sum3 : Sum  InputSameDT=on  SaturateOnIntegerOverflow=on  OutDataTypeStr=Inherit: Same as first input
  Sum4 : Sum  InputSameDT=on  SaturateOnIntegerOverflow=on  OutDataTypeStr=Inherit: Same as first input
  lce/lopt : Gain  Gain=1/loptHFL  SaturateOnIntegerOverflow=on  OutDataTypeStr=Inherit: Same as input  ParamDataTypeStr=Inherit: Same as input
  vmax*lopt : Gain  Gain=vmaxHFL*loptHFL  SaturateOnIntegerOverflow=on  OutDataTypeStr=Inherit: Same as input  ParamDataTypeStr=Inherit: Same as input
  Fmtc : Outport  InitialOutput=0  VectorParamsAs1DForOutWhenUnconnected=off
  Lce : Outport  Port=2  InitialOutput=0  VectorParamsAs1DForOutWhenUnconnected=off
  Vce : Outport  Port=3  InitialOutput=0  VectorParamsAs1DForOutWhenUnconnected=off
  Fce : Outport  Port=4  InitialOutput=0  VectorParamsAs1DForOutWhenUnconnected=off
  lse [m] : Outport  Port=5  InitialOutput=0  VectorParamsAs1DForOutWhenUnconnected=off
  wires:
  Integrator/1 -> Sum/2, lce/lopt/1, Lce/1  "lce"
  Sum/1 -> lse [m]/1, 1/lslack/1  "lse"
  lce/lopt/1 -> CE force-length relation/1(lce [lopt]), PE force-length relation/1(lce [lopt]), BE force-length relation/1(lce [lopt])
  Fv = Fse / (A*Fce)/1 -> "Fpe = F^*pe * fv "/1, CE inverse force-velocity relation/1(Fv[Fmax])  "fv"
  vmax*lopt/1 -> Integrator/1, Vce/1  "vce"
  lmtc [m]/1 -> Sum2/2, Sum/1  "lmtc"
  Fmax/1 -> Fmtc/1  "Fmtc"
  1/lslack/1 -> SE force-length relation/1(lse [lslack])
  SE force-length relation/1(fse [Fmax]) -> Fmax/1, Sum4/1
  Sum2/1 -> Integrator/2
  Constant/1 -> Sum2/1
  CE force-length relation/1(fce [Fmax]) -> 1/1
  PE force-length relation/1(fpe [Fmax]) -> "Fpe = F^*pe * fv "/2, Sum3/1
  1/1 -> Sum3/2
  BE force-length relation/1(fbe [Fmax]) -> Sum4/2
  Sum3/1 -> Fv = Fse / (A*Fce)/2
  CE inverse force-velocity relation/1(v[vmax]) -> vmax*lopt/1
  A/1 -> 1/2
  Sum4/1 -> Sum1/1, Fv = Fse / (A*Fce)/1  "Fse+Fbe"
  "Fpe = F^*pe * fv "/1 -> Sum1/2
  Sum1/1 -> Fmax1/1  "Fse+Fbe-Fpe"
  Fmax1/1 -> Fce/1

== system nms_sim_2D_cost/Muscle Actuation/L Ankle Joint Limits ==
  note: Ankle Joint Limits
  phi [rad] : Inport
  dphi [rad/s] : Inport  Port=2
  Gain1 : Gain  Gain=c_jointstop
  Gain2 : Gain  Gain=-1
  Gain3 : Gain  Gain=c_jointstop
  Gain4 : Gain  Gain=1/w_max_jointstop
  Limit Ankle Range : simulink/Logic and Bit Operations/Interval Test  Commented=on  IntervalClosedRight=on  uplimit=phi12_UpLimit + 40*pi/180  IntervalClosedLeft=on  lowlimit=phi12_LowLimit - 40*pi/180  OutDataTypeStr=boolean
  Logical Operator3 : Logic  Commented=on  Operator=NOT  AllPortsSameDT=off  OutDataTypeStr=boolean
  Mux1 : Mux  Inputs=2
  Mux3 : Mux  Inputs=2
  Overextension Torque : Fcn  Expr="- u(1)  *  (1-u(2)) * (u(2)<1) * (u(1)>0)"
  Overflexion Torque : Fcn  Expr="- u(1)  *  (1-u(2)) * (u(2)<1) * (u(1)<0)"
  Stop Simulation1 : Stop  Commented=on
  Sum : Sum  Inputs=|+-
  Sum1 : Sum  Inputs=|+-
  Sum2 : Sum
  overextension angle : Constant  Value=phi12_UpLimit
  overflexion angle : Constant  Value=phi12_LowLimit
  M_stop [Nm] : Outport  VectorParamsAs1DForOutWhenUnconnected=off
  wires:
  Mux3/1 -> Overextension Torque/1
  Gain3/1 -> Mux3/1
  dphi [rad/s]/1 -> Gain4/1
  overextension angle/1 -> Sum/2
  phi [rad]/1 -> Sum/1, Sum1/1, Limit Ankle Range/1
  Sum/1 -> Gain3/1
  Gain4/1 -> Gain2/1, Mux1/2
  Gain1/1 -> Mux1/1
  Sum1/1 -> Gain1/1
  overflexion angle/1 -> Sum1/2
  Mux1/1 -> Overflexion Torque/1
  Sum2/1 -> M_stop [Nm]/1
  Gain2/1 -> Mux3/2
  Overflexion Torque/1 -> Sum2/2
  Overextension Torque/1 -> Sum2/1
  Limit Ankle Range/1 -> Logical Operator3/1
  Logical Operator3/1 -> Stop Simulation1/1
